simulink model "My_gfm_battery_sil_1_PPC2"  (R2018b)
settings: Solver=ode45  StartTime=0.0  StopTime=30  MaxStep=1e-4  RelTol=1e-3
PreLoadFcn:
  | modelDir = fileparts(get_param(bdroot,'FileName'));
  | 
  | load_system(fullfile(modelDir,'controls_element_lib.slx'));
  | load_system(fullfile(modelDir,'test_sequence_lib.slx'));
InitFcn:
  | close all;
  | clear all;
  | clc;
  | 
  | % frequency nominals
  | F_NOM = 60;
  | W_NOM = 2 * pi * F_NOM;
  | 
  | % base values relative to inverter
  | % --------------------------------
  | VLL_INV_NOM = 480;
  | P_INV_NOM = 1e6;
  | Q_INV_NOM = 0.5e6;
  | S_INV_NOM = sqrt(P_INV_NOM^2 + Q_INV_NOM^2);
  | 
  | I_INV_BASE = S_INV_NOM/(sqrt(3)*VLL_INV_NOM);
  | Z_INV_BASE = VLL_INV_NOM^2/S_INV_NOM;
  | L_INV_BASE = Z_INV_BASE / W_NOM;
  | C_INV_BASE = 1 / (Z_INV_BASE * W_NOM);
  | 
  | % nominal ratings for power system model
  | % --------------------------------------
  | INVERTER_COUNT = 100;
  | 
  | VLV_NOM = VLL_INV_NOM;
  | VMV_NOM = 35e3;
  | VHV_NOM = 230e3;
  | S_PLANT = INVERTER_COUNT * S_INV_NOM;
  | 
  | N_GSU = VHV_NOM/VMV_NOM;
  | N_MVT = VMV_NOM/VLV_NOM;
  | 
  | I_LV_BASE = S_PLANT/(sqrt(3)*VLV_NOM);
  | I_MV_BASE = S_PLANT/(sqrt(3)*VMV_NOM);
  | I_HV_BASE = S_PLANT/(sqrt(3)*VHV_NOM);
  | 
  | Z_LV_BASE = VLV_NOM^2/S_PLANT;
  | Z_MV_BASE = VMV_NOM^2/S_PLANT;
  | Z_HV_BASE = VHV_NOM^2/S_PLANT;
  | 
  | L_LV_BASE = Z_LV_BASE / W_NOM;
  | L_MV_BASE = Z_MV_BASE / W_NOM;
  | L_HV_BASE = Z_HV_BASE / W_NOM;
  | C_LV_BASE = 1 / (Z_LV_BASE * W_NOM);
  | C_MV_BASE = 1 / (Z_MV_BASE * W_NOM);
  | C_HV_BASE = 1 / (Z_HV_BASE * W_NOM);
undefined symbols (not defined in the file): dQmax, dQmin, dVmax, dVmin, j, vmax, vmin
libraries: simulink x54, test_sequence_lib x22, controls_element_lib x9
(part 3 of 7)

== system My_gfm_battery_sil_1_PPC2/My Inverter Controller /My_currentSource_A ==
  note: S = sqrt(3)*V *conj(I)
      | P+jQ = sqrt(3)*(vd+jvq)*(id-jiq)
      | so P-jQ = sqrt(3)*(vd-jvq)*(id+jiq)
      | vq = 0, vd is LL RMS, id,iq are RMS
  note: S = sqrt(3) * VLL_rms * Irms
  note: RMS Id, Iq
  note: Vd+
  note: Why?
  note: RMS LL Pos Seq Voltage (Vd+, Vq+)
  note: Peak_Iabc
  note: cos x + j sin x
      | cos (x-120) + j (sin x -120)
      | cos (x+120) + j (sin x +120)
  enable : Inport
  P_request : Inport  Port=2
  Q_request : Inport  Port=3
  osc : Inport  Port=4
  Vpve : Inport  Port=5
  AND4 : Logic  IconShape=distinctive  AllPortsSameDT=off  OutDataTypeStr=boolean
  Complex to Real-Imag : ComplexToRealImag
  Conj : Math  Operator=conj  SaturateOnIntegerOverflow=on
  Constant : Constant  Value=0
  Constant2 : Constant  Value=CSOnline
  Divide : Product  Inputs=*/
  Gain : Gain  Gain=1/sqrt(3)
  Max1 : MinMax  Function=max  Inputs=2
  Real-Imag to Complex : RealImagToComplex
  Scope : Scope
  Switch : Switch  Criteria=u2 > Threshold
  Terminator : Terminator
  VLL_RATED : Constant  Value=VllRated
  current_modulator : Subsystem
  iref : Outport  VectorParamsAs1DForOutWhenUnconnected=on
  wires:
  Q_request/1 -> Real-Imag to Complex/2
  P_request/1 -> Real-Imag to Complex/1
  Complex to Real-Imag/1 -> Max1/1
  VLL_RATED/1 -> Max1/2
  Max1/1 -> Divide/2
  Divide/1 -> Gain/1
  Vpve/1 -> Complex to Real-Imag/1
  current_modulator/1(i_ref) -> Switch/1
  osc/1 -> current_modulator/2(osc)
  Real-Imag to Complex/1 -> Conj/1
  Conj/1 -> Divide/1
  Gain/1 -> Scope/1, current_modulator/1(I_cmd)
  Complex to Real-Imag/2 -> Terminator/1
  Constant/1 -> Switch/3
  Switch/1 -> iref/1
  Constant2/1 -> AND4/2
  AND4/1 -> Switch/2
  enable/1 -> AND4/1

== system My_gfm_battery_sil_1_PPC2/My Inverter Controller /My_machineModel_A ==
  note: Assume circuit controls will achieve
      | Iref = Imeas in the freq range of interest
  note: Measured terminal voltage
  note: Aligning with Rotor Frame
      | cos x + j sin x
      | cos (x-120) + j (sin x -120)
      | cos (x+120) + j (sin x +120)
  note: Peak Va, Vb, Vc
  note: RMS LL Vd
  note: RMS LL Vq
  Ex_Vref : Inport
  PLL_Vpve : Inport  Port=2
  Prequest : Inport  Port=3
  Ex_Fref : Inport  Port=4
  PLL_Fref : Inport  Port=5
  v_terminal : Inport  Port=6
  enable : Inport  Port=7
  AND4 : Logic  IconShape=distinctive  AllPortsSameDT=off  OutDataTypeStr=boolean
  AVR : Subsystem  AncestorBlock=controls_element_lib/machineModel_A/excitation
  Complex to Real-Imag : ComplexToRealImag
  Constant1 : Constant  Value=FreqRefSel
  Constant2 : Constant  Value=MachOnline
  Constant3 : Constant  Value=VoltRefSel
  Exciter : Subsystem  AncestorBlock=controls_element_lib/machineModel_A/excitation
  Scope : Scope  NumInputPorts=3
  Scope1 : Scope  NumInputPorts=4
  Scope2 : Scope  NumInputPorts=4
  Switch : Switch  Criteria=u2 > Threshold
  Switch1 : Switch  Criteria=u2 > Threshold
  Terminator : Terminator
  governer : Subsystem
  impedance emulation : Subsystem
  power analyzer : Subsystem
  rotor model : Subsystem
  voltage analyzer : Subsystem
  rotor_freq : Outport  VectorParamsAs1DForOutWhenUnconnected=on
  iref : Outport  Port=2  VectorParamsAs1DForOutWhenUnconnected=on
  wires:
  Switch/1 -> governer/2(Fref)
  AND4/1 -> governer/3(enabled), AVR/3(enabled), impedance emulation/2(enable)
  voltage analyzer/1(Vd) -> Scope2/2, AVR/6(Vd)
  rotor model/2(f_rotor) -> Scope1/4, governer/6(f_rotor), Scope/1, rotor_freq/1  "f_rotor"
  voltage analyzer/2(Vq) -> governer/5(Vq), Scope2/3, AVR/7(Vq)
  v_terminal/1 -> Scope2/1, voltage analyzer/2(v_terminal), power analyzer/2(vac), Scope/3, impedance emulation/3(v_terminal)
  impedance emulation/1(i_ref) -> iref/1, AVR/5(iac), power analyzer/1(iac)
  Prequest/1 -> governer/1(Prequest)
  governer/1(power) -> Scope1/1, rotor model/1(p_mechanical)
  Exciter/1(v_emf) -> Scope/2, impedance emulation/1(v_emf)  "v_emf"
  power analyzer/1(P) -> Scope1/2, rotor model/2(p_electrical)  "p_electrical"
  rotor model/1(osc[3]) -> voltage analyzer/1(osc[3]), Exciter/2(osc[3]), AVR/4(osc[3])
  power analyzer/2(Q) -> Scope1/3, AVR/2(Q)
  voltage analyzer/3(Vt_Mag) -> governer/4(Vt), Scope2/4
  Constant1/1 -> Switch/2
  Ex_Fref/1 -> Switch/1
  PLL_Fref/1 -> Switch/3
  Constant2/1 -> AND4/2
  enable/1 -> AND4/1
  AVR/1(Vexc) -> Exciter/1(Vexc)
  Ex_Vref/1 -> Switch1/1
  Constant3/1 -> Switch1/2
  Switch1/1 -> AVR/1(VRef)
  Complex to Real-Imag/1 -> Switch1/3
  Complex to Real-Imag/2 -> Terminator/1
  PLL_Vpve/1 -> Complex to Real-Imag/1

== system My_gfm_battery_sil_1_PPC2/My Inverter Controller /My_machineModel_A1 ==
  note: Assume circuit controls will achieve
      | Iref = Imeas in the freq range of interest
  note: Measured terminal voltage
  note: Aligning with Rotor Frame
      | cos x + j sin x
      | cos (x-120) + j (sin x -120)
      | cos (x+120) + j (sin x +120)
  note: Peak Va, Vb, Vc
  note: RMS LL Vd
  note: RMS LL Vq
  Vref : Inport
  Prequest : Inport  Port=2
  Ex_Fref : Inport  Port=3
  PLL_Fref : Inport  Port=4
  v_terminal : Inport  Port=5
  enable : Inport  Port=6
  AND4 : Logic  IconShape=distinctive  AllPortsSameDT=off  OutDataTypeStr=boolean
  Constant1 : Constant  Value=FreqRefSel
  Constant2 : Constant  Value=MachOnline
  Scope : Scope  NumInputPorts=3
  Scope1 : Scope  NumInputPorts=4
  Scope2 : Scope  NumInputPorts=4
  Switch : Switch  Criteria=u2 > Threshold
  Terminator : Terminator
  excitation : Subsystem  AncestorBlock=controls_element_lib/machineModel_A/excitation
  governer : Subsystem
  governer1 : Subsystem  Commented=on
  impedance emulation : Subsystem
  power analyzer : Subsystem
  rotor model : Subsystem
  voltage analyzer : Subsystem
  rotor_freq : Outport  VectorParamsAs1DForOutWhenUnconnected=on
  iref : Outport  Port=2  VectorParamsAs1DForOutWhenUnconnected=on
  wires:
  Vref/1 -> excitation/1(VRef)
  Switch/1 -> governer/2(Fref)
  AND4/1 -> governer/3(enabled), impedance emulation/2(enable)
  voltage analyzer/1(Vd) -> Scope2/2
  rotor model/2(f_rotor) -> Scope1/4, governer/6(f_rotor), Scope/1, rotor_freq/1  "f_rotor"
  voltage analyzer/2(Vq) -> governer/5(Vq), Scope2/3
  v_terminal/1 -> Scope2/1, voltage analyzer/2(v_terminal), power analyzer/2(vac), Scope/3, impedance emulation/3(v_terminal)
  impedance emulation/1(i_ref) -> iref/1, power analyzer/1(iac)
  Prequest/1 -> governer/1(Prequest)
  governer/1(power) -> Scope1/1, rotor model/1(p_mechanical)
  excitation/1(v_emf) -> Scope/2, impedance emulation/1(v_emf)  "v_emf"
  power analyzer/1(P) -> Scope1/2, rotor model/2(p_electrical)  "p_electrical"
  rotor model/1(osc[3]) -> excitation/2(osc[3]), voltage analyzer/1(osc[3])
  power analyzer/2(Q) -> Scope1/3, Terminator/1
  voltage analyzer/3(Vt_Mag) -> excitation/3(Vt), governer/4(Vt), Scope2/4
  Constant1/1 -> Switch/2
  Ex_Fref/1 -> Switch/1
  PLL_Fref/1 -> Switch/3
  Constant2/1 -> AND4/2
  enable/1 -> AND4/1

== system My_gfm_battery_sil_1_PPC2/My Inverter Controller /My_powerLimiter_A ==
  note: Why not using Vpve
  note: RMS_Id
  note: Peak_Iabc
  note: Power Limits from Battery Management system
  note: Ref current (Machine + Current source)
  note: cos x + j sin x
      | cos (x-120) + j (sin x -120)
      | cos (x+120) + j (sin x +120)
  i_ac : Inport
  v_ac : Inport  Port=2
  osc : Inport  Port=3
  P_lim_high : Inport  Port=4
  P_lim_low : Inport  Port=5
  Gain1 : Gain  Gain=1/(VllRated * sqrt(3))
  Product : Product
  Saturation Dynamic : simulink/Discontinuities/Saturation Dynamic  OutMin=[]  OutMax=[]  OutDataTypeStr=Inherit: Same as second input  OutDataType=fixdt(1, 16)  OutScaling=2^-10  DoSatur=off
  Sum of Elements : Sum  Inputs=+
  Sum1 : Sum  Inputs=|+-
  Transfer Fcn : TransferFcn  Denominator=[1/wPowerLimiter, 1]
  current_modulator : controls_element_lib/currentSource_A/current_modulator  SystemSampleTime=-1
  i_excess : Outport  VectorParamsAs1DForOutWhenUnconnected=on
  wires:
  Transfer Fcn/1 -> Sum1/1, Saturation Dynamic/2  "P_lpf"
  current_modulator/1 -> i_excess/1
  Saturation Dynamic/1 -> Sum1/2
  P_lim_low/1 -> Saturation Dynamic/3
  P_lim_high/1 -> Saturation Dynamic/1
  Sum1/1 -> Gain1/1
  Sum of Elements/1 -> Transfer Fcn/1  "P_inst"
  Gain1/1 -> current_modulator/1
  osc/1 -> current_modulator/2
  Product/1 -> Sum of Elements/1
  i_ac/1 -> Product/1
  v_ac/1 -> Product/2

== system My_gfm_battery_sil_1_PPC2/Plant Controller A1/Active Power Controller ==
  e : Inport
  en : Inport  Port=2
  Hold : Inport  Port=3
  Constant : Constant  Value=Pmax
  Constant1 : Constant  Value=0
  Constant2 : Constant  Value=Pmin
  Constant3 : Constant  Value=0
  Gain : Gain  Gain=Kpg
  Gain1 : Gain  Gain=Kig
  Integrator1 : Integrator  ExternalReset=level
  Logical Operator : Logic  Operator=OR  AllPortsSameDT=off  OutDataTypeStr=boolean
  OR : Logic  Operator=OR  AllPortsSameDT=off  OutDataTypeStr=boolean
  Relational Operator : RelationalOperator  Operator=>  OutDataTypeStr=boolean  RndMeth=Simplest
  Relational Operator1 : RelationalOperator  Operator=<  OutDataTypeStr=boolean  RndMeth=Simplest
  Saturation Dynamic : simulink/Discontinuities/Saturation Dynamic  OutMin=[]  OutMax=[]  OutDataTypeStr=Inherit: Same as second input  OutDataType=fixdt(1, 16)  OutScaling=2^-10  DoSatur=off
  Sum1 : Sum  Inputs=++|
  Switch1 : Switch  Criteria=u2 > Threshold
  Switch2 : Switch  Criteria=u2 > Threshold
  u : Outport
  wires:
  OR/1 -> Switch1/2
  Logical Operator/1 -> OR/2
  Constant2/1 -> Relational Operator1/2, Saturation Dynamic/3
  Sum1/1 -> Relational Operator1/1, Relational Operator/1, Saturation Dynamic/2
  Saturation Dynamic/1 -> u/1  "u"
  Gain1/1 -> Switch1/3
  Constant/1 -> Relational Operator/2, Saturation Dynamic/1
  Constant1/1 -> Switch1/1
  e/1 -> Gain1/1, Gain/1  "e"
  Gain/1 -> Switch2/3
  Relational Operator/1 -> Logical Operator/1
  Relational Operator1/1 -> Logical Operator/2
  Constant3/1 -> Switch2/1
  Hold/1 -> Switch2/2, OR/1
  Switch2/1 -> Sum1/1
  Switch1/1 -> Integrator1/1
  en/1 -> Integrator1/2
  Integrator1/1 -> Sum1/2

== system My_gfm_battery_sil_1_PPC2/Plant Controller A1/LVRT_foldback ==
  note: Delay the Power ramping after voltage drop
  Vpve_pu : Inport
  Abs : Abs
  Constant1 : Constant  Value=Pmax
  Constant2 : Constant  Value=-Pmin
  Gain : Gain  Gain=5
  LPF : Subsystem
  MinMax : MinMax  Function=max  Inputs=2
  Saturation : Saturate  UpperLimit=1  LowerLimit=0.05
  Sum1 : Sum  Inputs=|+-
  Sum2 : Sum  Inputs=|++
  assymmetric filter : Subsystem
  foldback_threshold : Constant  Value=Vfrz
  limit_pu : Outport  VectorParamsAs1DForOutWhenUnconnected=on
  wires:
  Sum1/1 -> LPF/1(in)
  Gain/1 -> Sum2/1
  LPF/1(out) -> Gain/1
  Sum2/1 -> Saturation/1
  foldback_threshold/1 -> Sum1/2
  Saturation/1 -> limit_pu/1
  assymmetric filter/1(out) -> Sum1/1
  Abs/1 -> assymmetric filter/1(in)
  Vpve_pu/1 -> Abs/1
  MinMax/1 -> Sum2/2
  Constant1/1 -> MinMax/1
  Constant2/1 -> MinMax/2

== system My_gfm_battery_sil_1_PPC2/Plant Controller A1/Line drop Compensation ==
  I : Inport
  V : Inport  Port=2
  Complex to Magnitude : ComplexToMagnitudeAngle  Output=Magnitude
  Gain : Gain  Gain=Rc
  Gain1 : Gain  Gain=j*Xc
  Sum : Sum  Inputs=|++
  Sum1 : Sum  Inputs=|-+
  Ve : Outport
  wires:
  I/1 -> Gain/1, Gain1/1
  Gain/1 -> Sum/1
  V/1 -> Sum1/2
  Sum/1 -> Sum1/1
  Gain1/1 -> Sum/2
  Sum1/1 -> Complex to Magnitude/1
  Complex to Magnitude/1 -> Ve/1  "Ve"

== system My_gfm_battery_sil_1_PPC2/Plant Controller A1/Meter ==
  note: in pu:
      | S = V * conj(I)
  note: RMS LL Pos Seq Voltage (Vd+, Vq+)
  note: RMS Pos Seq Current (Id+, Iq+)
  v : Inport
  i : Inport  Port=2
  Conj : Math  Operator=conj  SaturateOnIntegerOverflow=on
  PLL-analog : Subsystem
  Product : Product
  Sum of Elements : Sum  Inputs=+
  Terminator1 : Terminator
  Terminator2 : Terminator
  phasor_analysis : Subsystem
  phasor_analysis1 : Subsystem
  Vpve : Outport  VectorParamsAs1DForOutWhenUnconnected=on
  ipve : Outport  Port=2  VectorParamsAs1DForOutWhenUnconnected=on
  S : Outport  Port=3  VectorParamsAs1DForOutWhenUnconnected=on
  freq : Outport  Port=4  VectorParamsAs1DForOutWhenUnconnected=on
  wires:
  v/1 -> PLL-analog/1(ref), phasor_analysis/1(in)
  PLL-analog/1(freq) -> freq/1
  PLL-analog/2(osc) -> phasor_analysis1/2(osc), phasor_analysis/2(osc)
  i/1 -> phasor_analysis1/1(in)
  Conj/1 -> Product/2
  phasor_analysis/2(nve) -> Terminator1/1
  phasor_analysis1/2(nve) -> Terminator2/1
  phasor_analysis1/1(pve) -> ipve/1, Conj/1
  phasor_analysis/1(pve) -> Product/1, Vpve/1
  Product/1 -> Sum of Elements/1
  Sum of Elements/1 -> S/1

== system My_gfm_battery_sil_1_PPC2/Plant Controller A1/P  LPF ==
  note: disable integrator and pass through signal if tau is zero
  u : Inport
  Constant : Constant  Value=Tp
  Gain1 : Gain  Gain=1/(Tp+eps)  SaturateOnIntegerOverflow=on  OutDataTypeStr=Inherit: Same as input  ParamDataTypeStr=Inherit: Same as input
  Integrator : Integrator  UpperSaturationLimit=vmax  LowerSaturationLimit=vmin
  Sum : Sum  Inputs=|+-  SaturateOnIntegerOverflow=on  InputSameDT=on  OutDataTypeStr=Inherit: Same as first input
  Switch : Switch  Criteria=u2 > Threshold
  Switch1 : Switch  Criteria=u2 > Threshold
  y : Outport
  wires:
  u/1 -> Switch1/3, Sum/1
  Switch/1 -> Integrator/1
  Integrator/1 -> Sum/2, Switch1/1
  Constant/1 -> Switch/3, Switch1/2, Switch/2
  Sum/1 -> Gain1/1
  Switch1/1 -> y/1
  Gain1/1 -> Switch/1

== system My_gfm_battery_sil_1_PPC2/Plant Controller A1/P Lag LPF ==
  note: disable integrator and pass through signal if tau is zero
  u : Inport
  Constant : Constant  Value=Tlag
  Gain1 : Gain  Gain=1/(Tlag+eps)  SaturateOnIntegerOverflow=on  OutDataTypeStr=Inherit: Same as input  ParamDataTypeStr=Inherit: Same as input
  Integrator : Integrator  UpperSaturationLimit=vmax  LowerSaturationLimit=vmin
  Sum : Sum  Inputs=|+-  SaturateOnIntegerOverflow=on  InputSameDT=on  OutDataTypeStr=Inherit: Same as first input
  Switch : Switch  Criteria=u2 > Threshold
  Switch1 : Switch  Criteria=u2 > Threshold
  y : Outport
  wires:
  u/1 -> Switch1/3, Sum/1
  Switch/1 -> Integrator/1
  Integrator/1 -> Sum/2, Switch1/1
  Constant/1 -> Switch/3, Switch1/2, Switch/2
  Sum/1 -> Gain1/1
  Switch1/1 -> y/1
  Gain1/1 -> Switch/1

== system My_gfm_battery_sil_1_PPC2/Plant Controller A1/Q LPF ==
  note: disable integrator and pass through signal if tau is zero
  u : Inport
  Constant : Constant  Value=Tfltr
  Gain1 : Gain  Gain=1/(Tfltr+eps)  SaturateOnIntegerOverflow=on  OutDataTypeStr=Inherit: Same as input  ParamDataTypeStr=Inherit: Same as input
  Integrator : Integrator  UpperSaturationLimit=vmax  LowerSaturationLimit=vmin
  Sum : Sum  Inputs=|+-  SaturateOnIntegerOverflow=on  InputSameDT=on  OutDataTypeStr=Inherit: Same as first input
  Switch : Switch  Criteria=u2 > Threshold
  Switch1 : Switch  Criteria=u2 > Threshold
  y : Outport
  wires:
  u/1 -> Switch1/3, Sum/1
  Switch/1 -> Integrator/1
  Integrator/1 -> Sum/2, Switch1/1
  Constant/1 -> Switch/3, Switch1/2, Switch/2
  Sum/1 -> Gain1/1
  Switch1/1 -> y/1
  Gain1/1 -> Switch/1

== system My_gfm_battery_sil_1_PPC2/Plant Controller A1/Q Lead Lag ==
  note: disable integrator and pass through signal if tb is zero
  u : Inport
  Constant : Constant  Value=Tfv
  Gain : Gain  Gain=1/(Tfv+eps)
  Gain1 : Gain  Gain=Tft
  Integrator : Integrator
  Sum : Sum  Inputs=|+-
  Sum1 : Sum  Inputs=++|
  Switch : Switch  Criteria=u2 > Threshold
  Switch1 : Switch  Criteria=u2 > Threshold
  y : Outport
  wires:
  Sum1/1 -> Switch1/1
  Constant/1 -> Switch1/2, Switch/3, Switch/2
  u/1 -> Switch1/3, Sum/1
  Switch1/1 -> y/1
  Gain/1 -> Switch/1, Gain1/1
  Integrator/1 -> Sum1/2, Sum/2
  Sum/1 -> Gain/1
  Gain1/1 -> Sum1/1
  Switch/1 -> Integrator/1

== system My_gfm_battery_sil_1_PPC2/Plant Controller A1/Reactive Power Controller ==
  e : Inport
  en : Inport  Port=2
  Hold : Inport  Port=3
  Constant : Constant  Value=Qmax
  Constant1 : Constant  Value=0
  Constant2 : Constant  Value=Qmin
  Gain : Gain  Gain=Kp
  Gain1 : Gain  Gain=Ki
  Integrator1 : Integrator  ExternalReset=level
  Logical Operator : Logic  Operator=OR  AllPortsSameDT=off  OutDataTypeStr=boolean
  OR : Logic  Operator=OR  AllPortsSameDT=off  OutDataTypeStr=boolean
  Relational Operator : RelationalOperator  Operator=>  OutDataTypeStr=boolean  RndMeth=Simplest
  Relational Operator1 : RelationalOperator  Operator=<  OutDataTypeStr=boolean  RndMeth=Simplest
  Saturation Dynamic : simulink/Discontinuities/Saturation Dynamic  OutMin=[]  OutMax=[]  OutDataTypeStr=Inherit: Same as second input  OutDataType=fixdt(1, 16)  OutScaling=2^-10  DoSatur=off
  Sum1 : Sum  Inputs=++|
  Switch1 : Switch  Criteria=u2 > Threshold
  u : Outport
  wires:
  OR/1 -> Switch1/2
  Logical Operator/1 -> OR/2
  Hold/1 -> OR/1
  Constant2/1 -> Relational Operator1/2, Saturation Dynamic/3
  Sum1/1 -> Relational Operator1/1, Relational Operator/1, Saturation Dynamic/2
  Saturation Dynamic/1 -> u/1  "u"
  Switch1/1 -> Integrator1/1
  Gain1/1 -> Switch1/3
  Integrator1/1 -> Sum1/2
  Constant/1 -> Relational Operator/2, Saturation Dynamic/1
  Constant1/1 -> Switch1/1
  e/1 -> Gain1/1, Gain/1  "e"
  Gain/1 -> Sum1/1
  Relational Operator/1 -> Logical Operator/1
  Relational Operator1/1 -> Logical Operator/2
  en/1 -> Integrator1/2

== system My_gfm_battery_sil_1_PPC2/Plant Controller A1/Vcomp LPF ==
  note: disable integrator and pass through signal if tau is zero
  u : Inport
  Constant : Constant  Value=Tfltr
  Gain1 : Gain  Gain=1/(Tfltr+eps)  SaturateOnIntegerOverflow=on  OutDataTypeStr=Inherit: Same as input  ParamDataTypeStr=Inherit: Same as input
  Integrator : Integrator  UpperSaturationLimit=vmax  LowerSaturationLimit=vmin
  Sum : Sum  Inputs=|+-  SaturateOnIntegerOverflow=on  InputSameDT=on  OutDataTypeStr=Inherit: Same as first input
  Switch : Switch  Criteria=u2 > Threshold
  Switch1 : Switch  Criteria=u2 > Threshold
  y : Outport
  wires:
  u/1 -> Switch1/3, Sum/1
  Switch/1 -> Integrator/1
  Integrator/1 -> Sum/2, Switch1/1
  Constant/1 -> Switch/3, Switch1/2, Switch/2
  Sum/1 -> Gain1/1
  Switch1/1 -> y/1
  Gain1/1 -> Switch/1

== system My_gfm_battery_sil_1_PPC2/Plant Controller A3/Active Power Controller ==
  e : Inport
  en : Inport  Port=2
  Hold : Inport  Port=3
  Constant : Constant  Value=Pmax
  Constant1 : Constant  Value=0
  Constant2 : Constant  Value=Pmin
  Constant3 : Constant  Value=0
  Gain : Gain  Gain=Kpg
  Gain1 : Gain  Gain=Kig
  Integrator1 : Integrator  ExternalReset=level
  Logical Operator : Logic  Operator=OR  AllPortsSameDT=off  OutDataTypeStr=boolean
  OR : Logic  Operator=OR  AllPortsSameDT=off  OutDataTypeStr=boolean
  Relational Operator : RelationalOperator  Operator=>  OutDataTypeStr=boolean  RndMeth=Simplest
  Relational Operator1 : RelationalOperator  Operator=<  OutDataTypeStr=boolean  RndMeth=Simplest
  Saturation Dynamic : simulink/Discontinuities/Saturation Dynamic  OutMin=[]  OutMax=[]  OutDataTypeStr=Inherit: Same as second input  OutDataType=fixdt(1, 16)  OutScaling=2^-10  DoSatur=off
  Sum1 : Sum  Inputs=++|
  Switch1 : Switch  Criteria=u2 > Threshold
  Switch2 : Switch  Criteria=u2 > Threshold
  u : Outport
  wires:
  OR/1 -> Switch1/2
  Logical Operator/1 -> OR/2
  Constant2/1 -> Relational Operator1/2, Saturation Dynamic/3
  Sum1/1 -> Relational Operator1/1, Relational Operator/1, Saturation Dynamic/2
  Saturation Dynamic/1 -> u/1  "u"
  Gain1/1 -> Switch1/3
  Constant/1 -> Relational Operator/2, Saturation Dynamic/1
  Constant1/1 -> Switch1/1
  e/1 -> Gain1/1, Gain/1  "e"
  Gain/1 -> Switch2/3
  Relational Operator/1 -> Logical Operator/1
  Relational Operator1/1 -> Logical Operator/2
  Constant3/1 -> Switch2/1
  Hold/1 -> Switch2/2, OR/1
  Switch2/1 -> Sum1/1
  Switch1/1 -> Integrator1/1
  en/1 -> Integrator1/2
  Integrator1/1 -> Sum1/2

== system My_gfm_battery_sil_1_PPC2/Plant Controller A3/Active Power Controller1 ==
  e : Inport
  UpperLim : Inport  Port=2
  LowerLim : Inport  Port=3
  en : Inport  Port=4
  Constant2 : Constant  Value=0
  Gain3 : Gain  Gain=100e-3
  Integrator1 : Integrator  ExternalReset=level
  Saturation Dynamic : simulink/Discontinuities/Saturation Dynamic  OutMin=[]  OutMax=[]  OutDataTypeStr=Inherit: Same as second input  OutDataType=fixdt(1, 16)  OutScaling=2^-10  DoSatur=off
  Scope3 : Scope  NumInputPorts=5
  Sum1 : Sum  Inputs=++|
  Sum2 : Sum  Inputs=|+-
  u : Outport
  wires:
  LowerLim/1 -> Scope3/2, Saturation Dynamic/3
  Sum1/1 -> Saturation Dynamic/2
  Saturation Dynamic/1 -> Scope3/3, Gain3/1, u/1  "u"
  Integrator1/1 -> Scope3/4, Sum1/2
  UpperLim/1 -> Scope3/1, Saturation Dynamic/1
  e/1 -> Scope3/5, Sum2/1  "e"
  Constant2/1 -> Sum1/1
  Sum2/1 -> Integrator1/1
  Gain3/1 -> Sum2/2
  en/1 -> Integrator1/2

== system My_gfm_battery_sil_1_PPC2/Plant Controller A3/Active Power Controller2 ==
  e : Inport
  UpperLim : Inport  Port=2
  LowerLim : Inport  Port=3
  en : Inport  Port=4
  Constant2 : Constant  Value=0
  Gain3 : Gain  Gain=100e-3
  Integrator1 : Integrator  ExternalReset=level
  Saturation Dynamic : simulink/Discontinuities/Saturation Dynamic  OutMin=[]  OutMax=[]  OutDataTypeStr=Inherit: Same as second input  OutDataType=fixdt(1, 16)  OutScaling=2^-10  DoSatur=off
  Scope3 : Scope  NumInputPorts=5
  Sum1 : Sum  Inputs=++|
  Sum2 : Sum  Inputs=|+-
  u : Outport
  wires:
  LowerLim/1 -> Scope3/2, Saturation Dynamic/3
  Sum1/1 -> Saturation Dynamic/2
  Saturation Dynamic/1 -> Scope3/3, Gain3/1, u/1  "u"
  Integrator1/1 -> Scope3/4, Sum1/2
  UpperLim/1 -> Scope3/1, Saturation Dynamic/1
  e/1 -> Scope3/5, Sum2/1  "e"
  Constant2/1 -> Sum1/1
  Sum2/1 -> Integrator1/1
  Gain3/1 -> Sum2/2
  en/1 -> Integrator1/2

== system My_gfm_battery_sil_1_PPC2/Plant Controller A3/LVRT_foldback ==
  note: Delay the Power ramping after voltage drop
  Vpve_pu : Inport
  Abs : Abs
  Constant1 : Constant  Value=Pmax
  Constant2 : Constant  Value=-Pmin
  Gain : Gain  Gain=5
  LPF : Subsystem
  MinMax : MinMax  Function=max  Inputs=2
  Saturation : Saturate  UpperLimit=1  LowerLimit=0.05
  Sum1 : Sum  Inputs=|+-
  Sum2 : Sum  Inputs=|++
  assymmetric filter : Subsystem
  foldback_threshold : Constant  Value=Vfrz
  limit_pu : Outport  VectorParamsAs1DForOutWhenUnconnected=on
  wires:
  Sum1/1 -> LPF/1(in)
  Gain/1 -> Sum2/1
  LPF/1(out) -> Gain/1
  Sum2/1 -> Saturation/1
  foldback_threshold/1 -> Sum1/2
  Saturation/1 -> limit_pu/1
  assymmetric filter/1(out) -> Sum1/1
  Abs/1 -> assymmetric filter/1(in)
  Vpve_pu/1 -> Abs/1
  MinMax/1 -> Sum2/2
  Constant1/1 -> MinMax/1
  Constant2/1 -> MinMax/2

== system My_gfm_battery_sil_1_PPC2/Plant Controller A3/Line drop Compensation ==
  I : Inport
  V : Inport  Port=2
  Complex to Magnitude : ComplexToMagnitudeAngle  Output=Magnitude
  Gain : Gain  Gain=Rc
  Gain1 : Gain  Gain=j*Xc
  Sum : Sum  Inputs=|++
  Sum1 : Sum  Inputs=|-+
  Ve : Outport
  wires:
  I/1 -> Gain/1, Gain1/1
  Gain/1 -> Sum/1
  V/1 -> Sum1/2
  Sum/1 -> Sum1/1
  Gain1/1 -> Sum/2
  Sum1/1 -> Complex to Magnitude/1
  Complex to Magnitude/1 -> Ve/1  "Ve"

== system My_gfm_battery_sil_1_PPC2/Plant Controller A3/Meter ==
  note: in pu:
      | S = V * conj(I)
  note: RMS LL Pos Seq Voltage (Vd+, Vq+)
  note: RMS Pos Seq Current (Id+, Iq+)
  v : Inport
  i : Inport  Port=2
  Conj : Math  Operator=conj  SaturateOnIntegerOverflow=on
  PLL-analog : Subsystem
  Product : Product
  Sum of Elements : Sum  Inputs=+
  Terminator1 : Terminator
  Terminator2 : Terminator
  phasor_analysis : Subsystem
  phasor_analysis1 : Subsystem
  Vpve : Outport  VectorParamsAs1DForOutWhenUnconnected=on
  ipve : Outport  Port=2  VectorParamsAs1DForOutWhenUnconnected=on
  S : Outport  Port=3  VectorParamsAs1DForOutWhenUnconnected=on
  freq : Outport  Port=4  VectorParamsAs1DForOutWhenUnconnected=on
  wires:
  v/1 -> PLL-analog/1(ref), phasor_analysis/1(in)
  PLL-analog/1(freq) -> freq/1
  PLL-analog/2(osc) -> phasor_analysis1/2(osc), phasor_analysis/2(osc)
  i/1 -> phasor_analysis1/1(in)
  Conj/1 -> Product/2
  phasor_analysis/2(nve) -> Terminator1/1
  phasor_analysis1/2(nve) -> Terminator2/1
  phasor_analysis1/1(pve) -> ipve/1, Conj/1
  phasor_analysis/1(pve) -> Product/1, Vpve/1
  Product/1 -> Sum of Elements/1
  Sum of Elements/1 -> S/1

== system My_gfm_battery_sil_1_PPC2/Plant Controller A3/P  LPF ==
  note: disable integrator and pass through signal if tau is zero
  u : Inport
  Constant : Constant  Value=Tp
  Gain1 : Gain  Gain=1/(Tp+eps)  SaturateOnIntegerOverflow=on  OutDataTypeStr=Inherit: Same as input  ParamDataTypeStr=Inherit: Same as input
  Integrator : Integrator  UpperSaturationLimit=vmax  LowerSaturationLimit=vmin
  Sum : Sum  Inputs=|+-  SaturateOnIntegerOverflow=on  InputSameDT=on  OutDataTypeStr=Inherit: Same as first input
  Switch : Switch  Criteria=u2 > Threshold
  Switch1 : Switch  Criteria=u2 > Threshold
  y : Outport
  wires:
  u/1 -> Switch1/3, Sum/1
  Switch/1 -> Integrator/1
  Integrator/1 -> Sum/2, Switch1/1
  Constant/1 -> Switch/3, Switch1/2, Switch/2
  Sum/1 -> Gain1/1
  Switch1/1 -> y/1
  Gain1/1 -> Switch/1

== system My_gfm_battery_sil_1_PPC2/Plant Controller A3/P Lag LPF ==
  note: disable integrator and pass through signal if tau is zero
  u : Inport
  Constant : Constant  Value=Tlag
  Gain1 : Gain  Gain=1/(Tlag+eps)  SaturateOnIntegerOverflow=on  OutDataTypeStr=Inherit: Same as input  ParamDataTypeStr=Inherit: Same as input
  Integrator : Integrator  UpperSaturationLimit=vmax  LowerSaturationLimit=vmin
  Sum : Sum  Inputs=|+-  SaturateOnIntegerOverflow=on  InputSameDT=on  OutDataTypeStr=Inherit: Same as first input
  Switch : Switch  Criteria=u2 > Threshold
  Switch1 : Switch  Criteria=u2 > Threshold
  y : Outport
  wires:
  u/1 -> Switch1/3, Sum/1
  Switch/1 -> Integrator/1
  Integrator/1 -> Sum/2, Switch1/1
  Constant/1 -> Switch/3, Switch1/2, Switch/2
  Sum/1 -> Gain1/1
  Switch1/1 -> y/1
  Gain1/1 -> Switch/1

== system My_gfm_battery_sil_1_PPC2/Plant Controller A3/Q LPF ==
  note: disable integrator and pass through signal if tau is zero
  u : Inport
  Constant : Constant  Value=Tfltr
  Gain1 : Gain  Gain=1/(Tfltr+eps)  SaturateOnIntegerOverflow=on  OutDataTypeStr=Inherit: Same as input  ParamDataTypeStr=Inherit: Same as input
  Integrator : Integrator  UpperSaturationLimit=vmax  LowerSaturationLimit=vmin
  Sum : Sum  Inputs=|+-  SaturateOnIntegerOverflow=on  InputSameDT=on  OutDataTypeStr=Inherit: Same as first input
  Switch : Switch  Criteria=u2 > Threshold
  Switch1 : Switch  Criteria=u2 > Threshold
  y : Outport
  wires:
  u/1 -> Switch1/3, Sum/1
  Switch/1 -> Integrator/1
  Integrator/1 -> Sum/2, Switch1/1
  Constant/1 -> Switch/3, Switch1/2, Switch/2
  Sum/1 -> Gain1/1
  Switch1/1 -> y/1
  Gain1/1 -> Switch/1

== system My_gfm_battery_sil_1_PPC2/Plant Controller A3/Q Lead Lag ==
  note: disable integrator and pass through signal if tb is zero
  u : Inport
  Constant : Constant  Value=Tfv
  Gain : Gain  Gain=1/(Tfv+eps)
  Gain1 : Gain  Gain=Tft
  Integrator : Integrator
  Sum : Sum  Inputs=|+-
  Sum1 : Sum  Inputs=++|
  Switch : Switch  Criteria=u2 > Threshold
  Switch1 : Switch  Criteria=u2 > Threshold
  y : Outport
  wires:
  Sum1/1 -> Switch1/1
  Constant/1 -> Switch1/2, Switch/3, Switch/2
  u/1 -> Switch1/3, Sum/1
  Switch1/1 -> y/1
  Gain/1 -> Switch/1, Gain1/1
  Integrator/1 -> Sum1/2, Sum/2
  Sum/1 -> Gain/1
  Gain1/1 -> Sum1/1
  Switch/1 -> Integrator/1

== system My_gfm_battery_sil_1_PPC2/Plant Controller A3/Reactive Power Controller ==
  e : Inport
  en : Inport  Port=2
  Hold : Inport  Port=3
  Constant : Constant  Value=Qmax
  Constant1 : Constant  Value=0
  Constant2 : Constant  Value=Qmin
  Gain : Gain  Gain=Kp
  Gain1 : Gain  Gain=Ki
  Integrator1 : Integrator  ExternalReset=level
  Logical Operator : Logic  Operator=OR  AllPortsSameDT=off  OutDataTypeStr=boolean
  OR : Logic  Operator=OR  AllPortsSameDT=off  OutDataTypeStr=boolean
  Relational Operator : RelationalOperator  Operator=>  OutDataTypeStr=boolean  RndMeth=Simplest
  Relational Operator1 : RelationalOperator  Operator=<  OutDataTypeStr=boolean  RndMeth=Simplest
  Saturation Dynamic : simulink/Discontinuities/Saturation Dynamic  OutMin=[]  OutMax=[]  OutDataTypeStr=Inherit: Same as second input  OutDataType=fixdt(1, 16)  OutScaling=2^-10  DoSatur=off
  Sum1 : Sum  Inputs=++|
  Switch1 : Switch  Criteria=u2 > Threshold
  u : Outport
  wires:
  OR/1 -> Switch1/2
  Logical Operator/1 -> OR/2
  Hold/1 -> OR/1
  Constant2/1 -> Relational Operator1/2, Saturation Dynamic/3
  Sum1/1 -> Relational Operator1/1, Relational Operator/1, Saturation Dynamic/2
  Saturation Dynamic/1 -> u/1  "u"
  Switch1/1 -> Integrator1/1
  Gain1/1 -> Switch1/3
  Integrator1/1 -> Sum1/2
  Constant/1 -> Relational Operator/2, Saturation Dynamic/1
  Constant1/1 -> Switch1/1
  e/1 -> Gain1/1, Gain/1  "e"
  Gain/1 -> Sum1/1
  Relational Operator/1 -> Logical Operator/1
  Relational Operator1/1 -> Logical Operator/2
  en/1 -> Integrator1/2

== system My_gfm_battery_sil_1_PPC2/Plant Controller A3/Vcomp LPF ==
  note: disable integrator and pass through signal if tau is zero
  u : Inport
  Constant : Constant  Value=Tfltr
  Gain1 : Gain  Gain=1/(Tfltr+eps)  SaturateOnIntegerOverflow=on  OutDataTypeStr=Inherit: Same as input  ParamDataTypeStr=Inherit: Same as input
  Integrator : Integrator  UpperSaturationLimit=vmax  LowerSaturationLimit=vmin
  Sum : Sum  Inputs=|+-  SaturateOnIntegerOverflow=on  InputSameDT=on  OutDataTypeStr=Inherit: Same as first input
  Switch : Switch  Criteria=u2 > Threshold
  Switch1 : Switch  Criteria=u2 > Threshold
  y : Outport
  wires:
  u/1 -> Switch1/3, Sum/1
  Switch/1 -> Integrator/1
  Integrator/1 -> Sum/2, Switch1/1
  Constant/1 -> Switch/3, Switch1/2, Switch/2
  Sum/1 -> Gain1/1
  Switch1/1 -> y/1
  Gain1/1 -> Switch/1

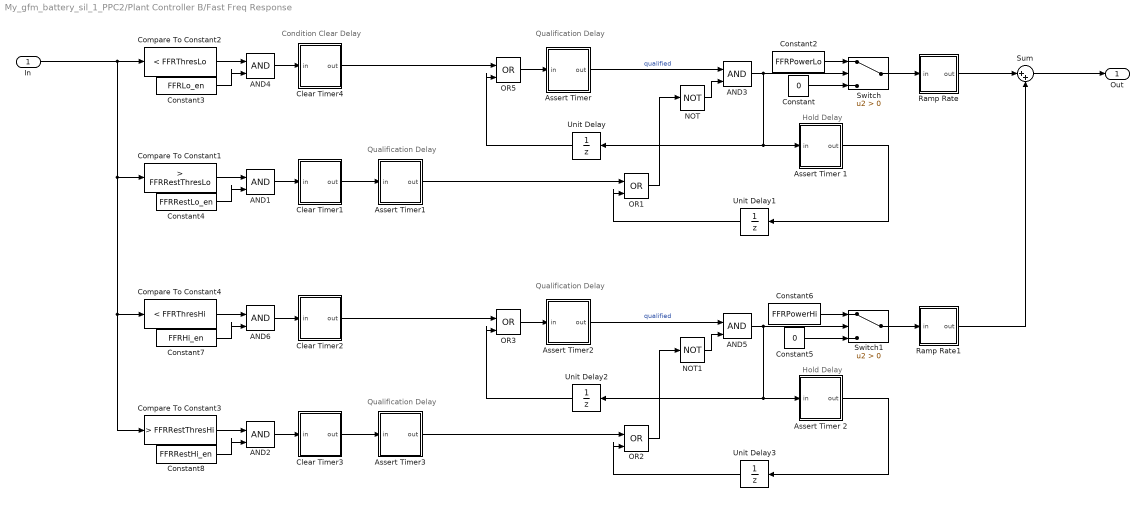
== system My_gfm_battery_sil_1_PPC2/Plant Controller B/Fast Freq Response ==
  note: Qualification Delay
  note: Hold Delay
  note: Qualification Delay
  note: Qualification Delay
  note: Hold Delay
  note: Qualification Delay
  note: Condition Clear Delay
  In : Inport
  AND{1..6} (6 alike) : Logic  IconShape=distinctive  AllPortsSameDT=off  OutDataTypeStr=boolean
  Assert Timer : Subsystem  mask{T_STEP=Ts, TIMEOUT=FFRTrigLoTime}
      mask prompts: T_STEP "Time step"
  Assert Timer 1 : Subsystem  mask{T_STEP=Ts, TIMEOUT=FFRHoldLoTime}
      mask prompts: T_STEP "Time step"
  Assert Timer 2 : Subsystem  mask{T_STEP=Ts, TIMEOUT=FFRHoldHiTime}
      mask prompts: T_STEP "Time step"
  Assert Timer1 : Subsystem  mask{T_STEP=Ts, TIMEOUT=FFRRestLoTime}
      mask prompts: T_STEP "Time step"
  Assert Timer2 : Subsystem  mask{T_STEP=Ts, TIMEOUT=FFRTrigHiTime}
      mask prompts: T_STEP "Time step"
  Assert Timer3 : Subsystem  mask{T_STEP=Ts, TIMEOUT=FFRRestHiTime}
      mask prompts: T_STEP "Time step"
  Clear Timer1 : Subsystem  mask{T_STEP=Ts, TIMEOUT=Time1, TIMER_INIT=0}
      mask prompts: T_STEP "Time step"; TIMER_INIT "Timer initial value"
  Clear Timer2 : Subsystem  mask{T_STEP=Ts, TIMEOUT=Time1, TIMER_INIT=0}
      mask prompts: T_STEP "Time step"; TIMER_INIT "Timer initial value"
  Clear Timer3 : Subsystem  mask{T_STEP=Ts, TIMEOUT=Time1, TIMER_INIT=0}
      mask prompts: T_STEP "Time step"; TIMER_INIT "Timer initial value"
  Clear Timer4 : Subsystem  mask{T_STEP=Ts, TIMEOUT=Time1, TIMER_INIT=0}
      mask prompts: T_STEP "Time step"; TIMER_INIT "Timer initial value"
  Compare To Constant1 : simulink/Logic and Bit Operations/Compare To Constant  relop=>  const=FFRRestThresLo  OutDataTypeStr=boolean
  Compare To Constant2 : simulink/Logic and Bit Operations/Compare To Constant  relop=<  const=FFRThresLo  OutDataTypeStr=boolean
  Compare To Constant3 : simulink/Logic and Bit Operations/Compare To Constant  relop=>  const=FFRRestThresHi  OutDataTypeStr=boolean
  Compare To Constant4 : simulink/Logic and Bit Operations/Compare To Constant  relop=<  const=FFRThresHi  OutDataTypeStr=boolean
  Constant : Constant  Value=0
  Constant2 : Constant  Value=FFRPowerLo
  Constant3 : Constant  Value=FFRLo_en
  Constant4 : Constant  Value=FFRRestLo_en
  Constant5 : Constant  Value=0
  Constant6 : Constant  Value=FFRPowerHi
  Constant7 : Constant  Value=FFRHi_en
  Constant8 : Constant  Value=FFRRestHi_en
  NOT : Logic  Operator=NOT  IconShape=distinctive  AllPortsSameDT=off  OutDataTypeStr=boolean
  NOT1 : Logic  Operator=NOT  IconShape=distinctive  AllPortsSameDT=off  OutDataTypeStr=boolean
  OR{1..3,5} (4 alike) : Logic  Operator=OR  IconShape=distinctive  AllPortsSameDT=off  OutDataTypeStr=boolean
  Ramp Rate : Subsystem  mask{T_STEP=Ts, UpRate=FFRLoRiseRate, DnRate=FFRLoFallRate}
      mask prompts: T_STEP "Time step"; UpRate "Rising Slew Rate"; DnRate "Falling Slew Rate"
  Ramp Rate1 : Subsystem  mask{T_STEP=Ts, UpRate=FFRHiRiseRate, DnRate=FFRHiFallRate}
      mask prompts: T_STEP "Time step"; UpRate "Rising Slew Rate"; DnRate "Falling Slew Rate"
  Sum : Sum  Inputs=|++
  Switch : Switch  Criteria=u2 > Threshold
  Switch1 : Switch  Criteria=u2 > Threshold
  Unit Delay{,1..3} (4 alike) : UnitDelay  SampleTime=Ts
  Out : Outport
  wires:
  Switch/1 -> Ramp Rate/1(in)
  Ramp Rate/1(out) -> Sum/1
  Constant/1 -> Switch/3
  AND3/1 -> Switch/2, Assert Timer 1/1(in), Unit Delay/1
  Clear Timer4/1(out) -> OR5/1
  OR1/1 -> NOT/1
  NOT/1 -> AND3/2
  OR5/1 -> Assert Timer/1(in)
  Unit Delay/1 -> OR5/2
  Assert Timer/1(out) -> AND3/1  "qualified"
  Compare To Constant2/1 -> AND4/1
  Constant3/1 -> AND4/2
  AND4/1 -> Clear Timer4/1(in)
  Unit Delay1/1 -> OR1/2
  Assert Timer 1/1(out) -> Unit Delay1/1
  Constant4/1 -> AND1/2
  AND1/1 -> Clear Timer1/1(in)
  Compare To Constant1/1 -> AND1/1
  Clear Timer1/1(out) -> Assert Timer1/1(in)
  Assert Timer1/1(out) -> OR1/1
  Constant2/1 -> Switch/1
  Sum/1 -> Out/1
  NOT1/1 -> AND5/2
  OR3/1 -> Assert Timer2/1(in)
  AND5/1 -> Switch1/2, Assert Timer 2/1(in), Unit Delay2/1
  Unit Delay3/1 -> OR2/2
  Unit Delay2/1 -> OR3/2
  Assert Timer 2/1(out) -> Unit Delay3/1
  Assert Timer2/1(out) -> AND5/1  "qualified"
  In/1 -> Compare To Constant3/1, Compare To Constant4/1, Compare To Constant1/1, Compare To Constant2/1
  Clear Timer3/1(out) -> Assert Timer3/1(in)
  OR2/1 -> NOT1/1
  Assert Timer3/1(out) -> OR2/1
  Clear Timer2/1(out) -> OR3/1
  Constant7/1 -> AND6/2
  Constant8/1 -> AND2/2
  AND2/1 -> Clear Timer3/1(in)
  Compare To Constant4/1 -> AND6/1
  Compare To Constant3/1 -> AND2/1
  AND6/1 -> Clear Timer2/1(in)
  Switch1/1 -> Ramp Rate1/1(in)
  Constant6/1 -> Switch1/1
  Constant5/1 -> Switch1/3
  Ramp Rate1/1(out) -> Sum/2

== system My_gfm_battery_sil_1_PPC2/Plant Controller B/LVRT_foldback ==
  note: Delay the Power ramping after voltage drop
  Vpve_pu : Inport
  Abs : Abs
  Constant1 : Constant  Value=Pmax
  Constant2 : Constant  Value=-Pmin
  Gain : Gain  Gain=5
  LPF : Subsystem
  MinMax : MinMax  Function=max  Inputs=2
  Saturation : Saturate  UpperLimit=1  LowerLimit=0.05
  Sum1 : Sum  Inputs=|+-
  Sum2 : Sum  Inputs=|++
  assymmetric filter : Subsystem
  foldback_threshold : Constant  Value=Vfrz
  limit_pu : Outport  VectorParamsAs1DForOutWhenUnconnected=on
  wires:
  Sum1/1 -> LPF/1(in)
  Gain/1 -> Sum2/1
  LPF/1(out) -> Gain/1
  Sum2/1 -> Saturation/1
  foldback_threshold/1 -> Sum1/2
  Saturation/1 -> limit_pu/1
  assymmetric filter/1(out) -> Sum1/1
  Abs/1 -> assymmetric filter/1(in)
  Vpve_pu/1 -> Abs/1
  MinMax/1 -> Sum2/2
  Constant1/1 -> MinMax/1
  Constant2/1 -> MinMax/2

== system My_gfm_battery_sil_1_PPC2/Plant Controller B/Meter ==
  note: in pu:
      | S = V * conj(I)
  note: RMS LL Pos Seq Voltage (Vd+, Vq+)
  note: RMS Pos Seq Current (Id+, Iq+)
  v : Inport
  i : Inport  Port=2
  Conj : Math  Operator=conj  SaturateOnIntegerOverflow=on
  PLL-analog : Subsystem
  Product : Product
  Sum of Elements : Sum  Inputs=+
  Terminator1 : Terminator
  Terminator2 : Terminator
  phasor_analysis : Subsystem
  phasor_analysis1 : Subsystem
  Vpve : Outport  VectorParamsAs1DForOutWhenUnconnected=on
  ipve : Outport  Port=2  VectorParamsAs1DForOutWhenUnconnected=on
  S : Outport  Port=3  VectorParamsAs1DForOutWhenUnconnected=on
  freq : Outport  Port=4  VectorParamsAs1DForOutWhenUnconnected=on
  wires:
  v/1 -> PLL-analog/1(ref), phasor_analysis/1(in)
  PLL-analog/1(freq) -> freq/1
  PLL-analog/2(osc) -> phasor_analysis1/2(osc), phasor_analysis/2(osc)
  i/1 -> phasor_analysis1/1(in)
  Conj/1 -> Product/2
  phasor_analysis/2(nve) -> Terminator1/1
  phasor_analysis1/2(nve) -> Terminator2/1
  phasor_analysis1/1(pve) -> ipve/1, Conj/1
  phasor_analysis/1(pve) -> Product/1, Vpve/1
  Product/1 -> Sum of Elements/1
  Sum of Elements/1 -> S/1

== system My_gfm_battery_sil_1_PPC2/Plant Controller B/P  LPF ==
  note: disable integrator and pass through signal if tau is zero
  u : Inport
  Constant : Constant  Value=Tp
  Gain1 : Gain  Gain=1/(Tp+eps)  SaturateOnIntegerOverflow=on  OutDataTypeStr=Inherit: Same as input  ParamDataTypeStr=Inherit: Same as input
  Integrator : Integrator  UpperSaturationLimit=vmax  LowerSaturationLimit=vmin
  Sum : Sum  Inputs=|+-  SaturateOnIntegerOverflow=on  InputSameDT=on  OutDataTypeStr=Inherit: Same as first input
  Switch : Switch  Criteria=u2 > Threshold
  Switch1 : Switch  Criteria=u2 > Threshold
  y : Outport
  wires:
  u/1 -> Switch1/3, Sum/1
  Switch/1 -> Integrator/1
  Integrator/1 -> Sum/2, Switch1/1
  Constant/1 -> Switch/3, Switch1/2, Switch/2
  Sum/1 -> Gain1/1
  Switch1/1 -> y/1
  Gain1/1 -> Switch/1

== system My_gfm_battery_sil_1_PPC2/Plant Controller B/P Lag LPF ==
  note: disable integrator and pass through signal if tau is zero
  u : Inport
  Constant : Constant  Value=Tlagp
  Gain1 : Gain  Gain=1/(Tlagp+eps)  SaturateOnIntegerOverflow=on  OutDataTypeStr=Inherit: Same as input  ParamDataTypeStr=Inherit: Same as input
  Integrator : Integrator  UpperSaturationLimit=vmax  LowerSaturationLimit=vmin
  Sum : Sum  Inputs=|+-  SaturateOnIntegerOverflow=on  InputSameDT=on  OutDataTypeStr=Inherit: Same as first input
  Switch : Switch  Criteria=u2 > Threshold
  Switch1 : Switch  Criteria=u2 > Threshold
  y : Outport
  wires:
  u/1 -> Switch1/3, Sum/1
  Switch/1 -> Integrator/1
  Integrator/1 -> Sum/2, Switch1/1
  Constant/1 -> Switch/3, Switch1/2, Switch/2
  Sum/1 -> Gain1/1
  Switch1/1 -> y/1
  Gain1/1 -> Switch/1

== system My_gfm_battery_sil_1_PPC2/Plant Controller B/PF LPF ==
  note: disable integrator and pass through signal if tau is zero
  u : Inport
  Constant : Constant  Value=Tpf
  Gain1 : Gain  Gain=1/(Tpf+eps)  SaturateOnIntegerOverflow=on  OutDataTypeStr=Inherit: Same as input  ParamDataTypeStr=Inherit: Same as input
  Integrator : Integrator  UpperSaturationLimit=vmax  LowerSaturationLimit=vmin
  Sum : Sum  Inputs=|+-  SaturateOnIntegerOverflow=on  InputSameDT=on  OutDataTypeStr=Inherit: Same as first input
  Switch : Switch  Criteria=u2 > Threshold
  Switch1 : Switch  Criteria=u2 > Threshold
  y : Outport
  wires:
  u/1 -> Switch1/3, Sum/1
  Switch/1 -> Integrator/1
  Integrator/1 -> Sum/2, Switch1/1
  Constant/1 -> Switch/3, Switch1/2, Switch/2
  Sum/1 -> Gain1/1
  Switch1/1 -> y/1
  Gain1/1 -> Switch/1

== system My_gfm_battery_sil_1_PPC2/Plant Controller B/Primary Freq Response ==
  In : Inport
  Gain1 : Gain  Gain=Kpfdn
  Gain2 : Gain  Gain=Kpfup
  Saturation1 : Saturate  UpperLimit=0  LowerLimit=-inf
  Saturation17 : Saturate  UpperLimit=Pfreqmax  LowerLimit=Pfreqmin
  Saturation2 : Saturate  UpperLimit=inf  LowerLimit=0
  Saturation4 : Saturate  UpperLimit=fdbd1  LowerLimit=fdbd2
  Sum4 : Sum  Inputs=++|
  Sum6 : Sum  Inputs=|+-
  f  LPF : Subsystem
  Out : Outport
  wires:
  Sum4/1 -> Saturation17/1
  Sum6/1 -> Gain2/1, Gain1/1
  Saturation4/1 -> Sum6/2
  Saturation17/1 -> f  LPF/1(u)
  Saturation2/1 -> Sum4/2
  Gain1/1 -> Saturation1/1
  Gain2/1 -> Saturation2/1
  In/1 -> Sum6/1, Saturation4/1
  Saturation1/1 -> Sum4/1
  f  LPF/1(y) -> Out/1

== system My_gfm_battery_sil_1_PPC2/Plant Controller B/Q LPF ==
  note: disable integrator and pass through signal if tau is zero
  u : Inport
  Constant : Constant  Value=Tfltr
  Gain1 : Gain  Gain=1/(Tfltr+eps)  SaturateOnIntegerOverflow=on  OutDataTypeStr=Inherit: Same as input  ParamDataTypeStr=Inherit: Same as input
  Integrator : Integrator  UpperSaturationLimit=vmax  LowerSaturationLimit=vmin
  Sum : Sum  Inputs=|+-  SaturateOnIntegerOverflow=on  InputSameDT=on  OutDataTypeStr=Inherit: Same as first input
  Switch : Switch  Criteria=u2 > Threshold
  Switch1 : Switch  Criteria=u2 > Threshold
  y : Outport
  wires:
  u/1 -> Switch1/3, Sum/1
  Switch/1 -> Integrator/1
  Integrator/1 -> Sum/2, Switch1/1
  Constant/1 -> Switch/3, Switch1/2, Switch/2
  Sum/1 -> Gain1/1
  Switch1/1 -> y/1
  Gain1/1 -> Switch/1

== system My_gfm_battery_sil_1_PPC2/Plant Controller B/Q Lead Lag ==
  note: disable integrator and pass through signal if tb is zero
  u : Inport
  Constant : Constant  Value=Tlagq
  Gain : Gain  Gain=1/(Tlagq+eps)
  Gain1 : Gain  Gain=Tleadq
  Integrator : Integrator
  Sum : Sum  Inputs=|+-
  Sum1 : Sum  Inputs=++|
  Switch : Switch  Criteria=u2 > Threshold
  Switch1 : Switch  Criteria=u2 > Threshold
  y : Outport
  wires:
  Sum1/1 -> Switch1/1
  Constant/1 -> Switch1/2, Switch/3, Switch/2
  u/1 -> Switch1/3, Sum/1
  Switch1/1 -> y/1
  Gain/1 -> Switch/1, Gain1/1
  Integrator/1 -> Sum1/2, Sum/2
  Sum/1 -> Gain/1
  Gain1/1 -> Sum1/1
  Switch/1 -> Integrator/1

== system My_gfm_battery_sil_1_PPC2/Plant Controller B/Ramp Rate ==
  in : Inport
  Constant1 : Constant  Value=UpRate
  Constant2 : Constant  Value=DnRate
  Constant4 : Constant  Value=T_STEP
  Product1 : Product
  Product2 : Product
  Saturation Dynamic : simulink/Discontinuities/Saturation Dynamic  OutMin=[]  OutMax=[]  OutDataTypeStr=Inherit: Same as second input  OutDataType=fixdt(1, 16)  OutScaling=2^-10  DoSatur=off
  Sum3 : Sum  Inputs=|++
  Sum4 : Sum  Inputs=|+-
  Unit Delay1 : UnitDelay  SampleTime=T_STEP
  out : Outport  VectorParamsAs1DForOutWhenUnconnected=on
  wires:
  Saturation Dynamic/1 -> Sum3/1
  Sum3/1 -> Unit Delay1/1, out/1
  Unit Delay1/1 -> Sum4/2, Sum3/2
  Sum4/1 -> Saturation Dynamic/2
  in/1 -> Sum4/1
  Constant1/1 -> Product1/2
  Constant4/1 -> Product2/1, Product1/1
  Product1/1 -> Saturation Dynamic/1
  Product2/1 -> Saturation Dynamic/3
  Constant2/1 -> Product2/2

== system My_gfm_battery_sil_1_PPC2/Plant Controller B/Ramp Rate1 ==
  in : Inport
  Constant1 : Constant  Value=UpRate
  Constant2 : Constant  Value=DnRate
  Constant4 : Constant  Value=T_STEP
  Product1 : Product
  Product2 : Product
  Saturation Dynamic : simulink/Discontinuities/Saturation Dynamic  OutMin=[]  OutMax=[]  OutDataTypeStr=Inherit: Same as second input  OutDataType=fixdt(1, 16)  OutScaling=2^-10  DoSatur=off
  Sum3 : Sum  Inputs=|++
  Sum4 : Sum  Inputs=|+-
  Unit Delay1 : UnitDelay  SampleTime=T_STEP
  out : Outport  VectorParamsAs1DForOutWhenUnconnected=on
  wires:
  Saturation Dynamic/1 -> Sum3/1
  Sum3/1 -> Unit Delay1/1, out/1
  Unit Delay1/1 -> Sum4/2, Sum3/2
  Sum4/1 -> Saturation Dynamic/2
  in/1 -> Sum4/1
  Constant1/1 -> Product1/2
  Constant4/1 -> Product2/1, Product1/1
  Product1/1 -> Saturation Dynamic/1
  Product2/1 -> Saturation Dynamic/3
  Constant2/1 -> Product2/2

== system My_gfm_battery_sil_1_PPC2/Plant Controller B/Subsystem ==
  note: (S^2/V^2) * R_col
  note: (S^2/V^2) * X_col
  Qcmd : Inport
  Pcmd : Inport  Port=2
  Vmag : Inport  Port=3
  Constant14 : Constant  Value=0.01
  Divide : Product  Inputs=*/
  Gain8 : Gain  Gain=Rc
  Gain9 : Gain  Gain=Xc
  Math Function : Math  Operator=square  SaturateOnIntegerOverflow=on
  Math Function1 : Math  Operator=square  SaturateOnIntegerOverflow=on
  MinMax : MinMax  Function=max  Inputs=2
  Sum11 : Sum  Inputs=++|
  Qloss : Outport
  Ploss : Outport  Port=2
  wires:
  Math Function1/1 -> Sum11/1
  Pcmd/1 -> Math Function/1
  Gain9/1 -> Qloss/1
  Math Function/1 -> Sum11/2
  Qcmd/1 -> Math Function1/1
  Divide/1 -> Gain9/1, Gain8/1
  Gain8/1 -> Ploss/1
  Vmag/1 -> MinMax/1
  Sum11/1 -> Divide/1
  MinMax/1 -> Divide/2
  Constant14/1 -> MinMax/2

== system My_gfm_battery_sil_1_PPC2/Plant Controller B/v LPF ==
  note: disable integrator and pass through signal if tau is zero
  u : Inport
  Constant : Constant  Value=Tpv
  Gain1 : Gain  Gain=1/(Tpv+eps)  SaturateOnIntegerOverflow=on  OutDataTypeStr=Inherit: Same as input  ParamDataTypeStr=Inherit: Same as input
  Integrator : Integrator  UpperSaturationLimit=vmax  LowerSaturationLimit=vmin
  Sum : Sum  Inputs=|+-  SaturateOnIntegerOverflow=on  InputSameDT=on  OutDataTypeStr=Inherit: Same as first input
  Switch : Switch  Criteria=u2 > Threshold
  Switch1 : Switch  Criteria=u2 > Threshold
  y : Outport
  wires:
  u/1 -> Switch1/3, Sum/1
  Switch/1 -> Integrator/1
  Integrator/1 -> Sum/2, Switch1/1
  Constant/1 -> Switch/3, Switch1/2, Switch/2
  Sum/1 -> Gain1/1
  Switch1/1 -> y/1
  Gain1/1 -> Switch/1

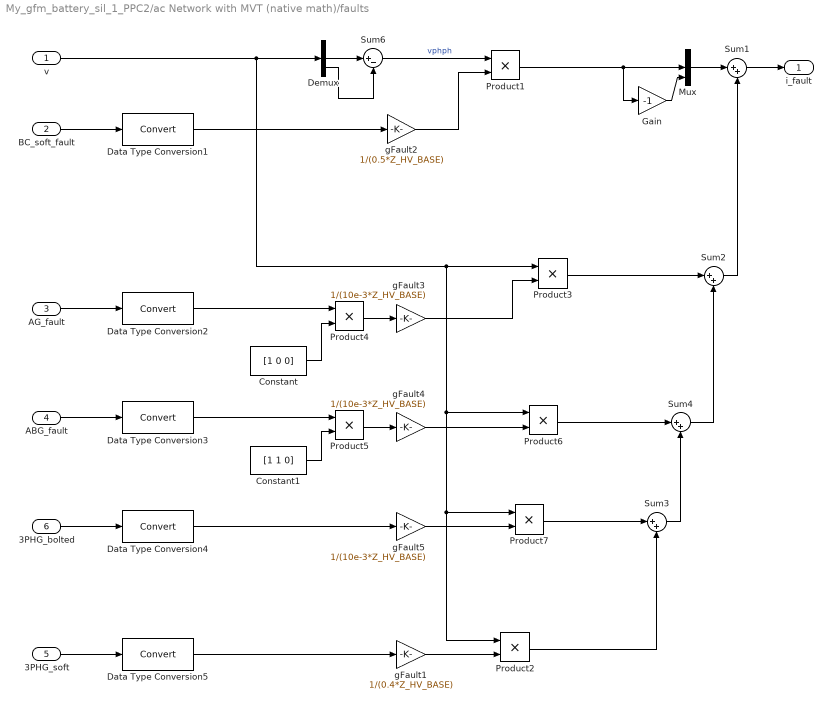
== system My_gfm_battery_sil_1_PPC2/ac Network with MVT (native math)/faults ==
  v : Inport
  BC_soft_fault : Inport  Port=2
  AG_fault : Inport  Port=3
  ABG_fault : Inport  Port=4
  3PHG_soft : Inport  Port=5
  3PHG_bolted : Inport  Port=6
  Constant : Constant  Value=[1 0 0]
  Constant1 : Constant  Value=[1 1 0]
  Data Type Conversion{1..5} (5 alike) : DataTypeConversion
  Demux : Demux  Outputs=3
  Gain : Gain  Gain=-1
  Mux : Mux  Inputs=3
  Product{1..7} (7 alike) : Product
  Sum{1..4} (4 alike) : Sum  Inputs=|++
  Sum6 : Sum  Inputs=|+-
  gFault1 : Gain  Gain=1/(0.4*Z_HV_BASE)
  gFault2 : Gain  Gain=1/(0.5*Z_HV_BASE)
  gFault3 : Gain  Gain=1/(10e-3*Z_HV_BASE)
  gFault4 : Gain  Gain=1/(10e-3*Z_HV_BASE)
  gFault5 : Gain  Gain=1/(10e-3*Z_HV_BASE)
  i_fault : Outport  VectorParamsAs1DForOutWhenUnconnected=on
  wires:
  Product2/1 -> Sum3/2
  gFault1/1 -> Product2/2
  Sum1/1 -> i_fault/1
  Product1/1 -> Gain/1, Mux/2
  v/1 -> Demux/1, Product3/1, Product6/1, Product7/1, Product2/1
  Demux/3 -> Sum6/2
  Demux/2 -> Sum6/1
  Gain/1 -> Mux/3
  Sum6/1 -> Product1/1  "vphph"
  gFault2/1 -> Product1/2
  gFault3/1 -> Product3/2
  Mux/1 -> Sum1/1
  Product4/1 -> gFault3/1
  Constant/1 -> Product4/2
  Constant1/1 -> Product5/2
  Product5/1 -> gFault4/1
  Product3/1 -> Sum2/1
  gFault4/1 -> Product6/2
  gFault5/1 -> Product7/2
  BC_soft_fault/1 -> Data Type Conversion1/1
  AG_fault/1 -> Data Type Conversion2/1
  ABG_fault/1 -> Data Type Conversion3/1
  3PHG_bolted/1 -> Data Type Conversion4/1
  3PHG_soft/1 -> Data Type Conversion5/1
  Sum2/1 -> Sum1/2
  Product6/1 -> Sum4/1
  Sum4/1 -> Sum2/2
  Product7/1 -> Sum3/1
  Sum3/1 -> Sum4/2
  Data Type Conversion1/1 -> gFault2/1
  Data Type Conversion2/1 -> Product4/1
  Data Type Conversion3/1 -> Product5/1
  Data Type Conversion4/1 -> gFault5/1
  Data Type Conversion5/1 -> gFault1/1

== system My_gfm_battery_sil_1_PPC2/ac Network with MVT (native math)/filter_caps ==
  i : Inport
  Gain1 : Gain  Gain=1/(0.03*C_LV_BASE)
  Integrator1 : Integrator
  v : Outport  VectorParamsAs1DForOutWhenUnconnected=on
  wires:
  Gain1/1 -> Integrator1/1
  Integrator1/1 -> v/1
  i/1 -> Gain1/1

== system My_gfm_battery_sil_1_PPC2/ac Network with MVT (native math)/filter_inductors ==
  v : Inport
  en : Inport  Port=2
  Gain1 : Gain  Gain=1/(0.02*L_LV_BASE)
  Integrator1 : Integrator  ExternalReset=level
  NOT : Logic  Operator=NOT  IconShape=distinctive  AllPortsSameDT=off  OutDataTypeStr=boolean
  i : Outport  VectorParamsAs1DForOutWhenUnconnected=on
  wires:
  NOT/1 -> Integrator1/2
  v/1 -> Gain1/1
  Integrator1/1 -> i/1
  Gain1/1 -> Integrator1/1
  en/1 -> NOT/1

== system My_gfm_battery_sil_1_PPC2/ac Network with MVT (native math)/solver_LPF ==
  In1 : Inport
  Gain : Gain  Gain=1/50e-6
  Integrator1 : Integrator
  Sum1 : Sum  Inputs=|+-
  Out1 : Outport  VectorParamsAs1DForOutWhenUnconnected=on
  wires:
  Gain/1 -> Integrator1/1
  Sum1/1 -> Gain/1
  Integrator1/1 -> Out1/1, Sum1/2
  In1/1 -> Sum1/1

== system My_gfm_battery_sil_1_PPC2/ac Network with MVT (native math)/solver_LPF1 ==
  In1 : Inport
  Gain : Gain  Gain=1/1e-3
  Integrator1 : Integrator
  Sum1 : Sum  Inputs=|+-
  Out1 : Outport  VectorParamsAs1DForOutWhenUnconnected=on
  wires:
  In1/1 -> Sum1/1
  Integrator1/1 -> Sum1/2, Out1/1
  Sum1/1 -> Gain/1
  Gain/1 -> Integrator1/1

== system My_gfm_battery_sil_1_PPC2/ac Network with MVT (native math)/solver_LPF3 ==
  In1 : Inport
  Gain : Gain  Gain=1/50e-6
  Integrator1 : Integrator
  Sum1 : Sum  Inputs=|+-
  Out1 : Outport  VectorParamsAs1DForOutWhenUnconnected=on
  wires:
  Gain/1 -> Integrator1/1
  Sum1/1 -> Gain/1
  Integrator1/1 -> Out1/1, Sum1/2
  In1/1 -> Sum1/1

== system My_gfm_battery_sil_1_PPC2/AcMeter1/PLL_3ph/SOGI ==
  in : Inport
  fnom : Inport  Port=2
  2pi : Gain  Gain=2*pi
  Integrator2 : Integrator
  Integrator3 : Integrator
  Product : Product
  Product1 : Product
  Sum4 : Sum  Inputs=|+-
  Sum5 : Sum  Inputs=|+-
  alpha : Gain  Gain=0.1
  notch : Outport  VectorParamsAs1DForOutWhenUnconnected=on
  bpf : Outport  Port=2  VectorParamsAs1DForOutWhenUnconnected=on
  wires:
  in/1 -> Sum5/1
  fnom/1 -> 2pi/1
  Integrator2/1 -> Product1/1, Sum5/2, bpf/1
  alpha/1 -> Sum4/1
  Sum5/1 -> alpha/1, notch/1
  Sum4/1 -> Product/1
  Integrator3/1 -> Sum4/2
  2pi/1 -> Product1/2, Product/2
  Product/1 -> Integrator2/1
  Product1/1 -> Integrator3/1

== system My_gfm_battery_sil_1_PPC2/AcMeter1/PLL_3ph/oscillator_3ph ==
  f : Inport
  Cos : Trigonometry  Operator=cos
  Gain : Gain  Gain=2*pi
  Integrator : Integrator
  Real-Imag to Complex : RealImagToComplex
  Sin : Trigonometry
  Sum1 : Sum  Inputs=|++
  phase_shift : Constant  Value=[0 -1/3 -2/3]
  osc[3] : Outport  VectorParamsAs1DForOutWhenUnconnected=on
  wires:
  f/1 -> Integrator/1
  Real-Imag to Complex/1 -> osc[3]/1
  Cos/1 -> Real-Imag to Complex/1
  Gain/1 -> Cos/1, Sin/1
  Integrator/1 -> Sum1/1
  Sin/1 -> Real-Imag to Complex/2
  phase_shift/1 -> Sum1/2
  Sum1/1 -> Gain/1

== system My_gfm_battery_sil_1_PPC2/AcMeter1/phasor_analysis/complex_LPF1 ==
  In1 : Inport
  Complex to Real-Imag : ComplexToRealImag
  Integrator : Integrator
  Integrator1 : Integrator
  Real-Imag to Complex : RealImagToComplex
  Sum1 : Sum  Inputs=|+-
  Sum2 : Sum  Inputs=|+-
  wLPF : Gain  Gain=wLPF
  wLPF1 : Gain  Gain=wLPF
  1 : Outport  VectorParamsAs1DForOutWhenUnconnected=on
  wires:
  Complex to Real-Imag/2 -> Sum2/1
  Sum2/1 -> wLPF1/1
  wLPF1/1 -> Integrator1/1
  Integrator1/1 -> Sum2/2, Real-Imag to Complex/2
  Real-Imag to Complex/1 -> 1/1
  In1/1 -> Complex to Real-Imag/1
  Integrator/1 -> Real-Imag to Complex/1, Sum1/2
  wLPF/1 -> Integrator/1
  Sum1/1 -> wLPF/1
  Complex to Real-Imag/1 -> Sum1/1
